simulink library "MK_SZ"  (R2026a)
settings: Solver=VariableStepAuto
settings Model: Creator=Szalay  LastModifiedBy=Szalay

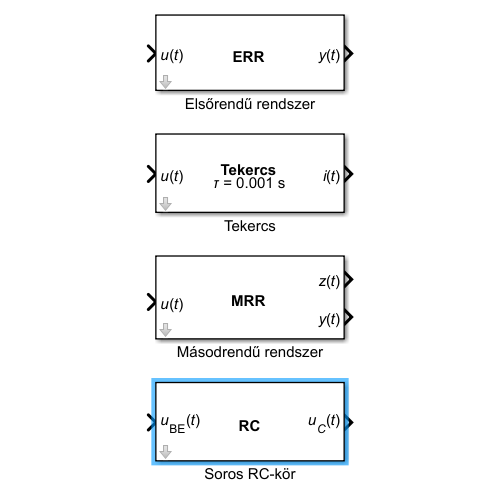
[thumbnail: Simulink's stored preview of the top-level diagram]
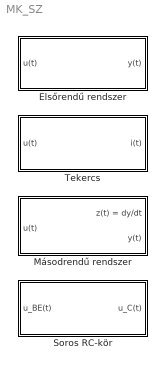
== system MK_SZ ==
  Elsőrendű rendszer : Subsystem  mask(Elsőrendű rendszer){K=1, tau=1, y_0=0}
      mask prompts: K "Állandósult állapoti erősítés"; tau "Időállandó (s)"; y_0 "A kimenet kezdeti értéke"
      mask help: A lineáris elsőrendű rendszer modellje.
      mask DialogControl ParameterGroupVar Prompt: Rendszerparaméterek
      mask DialogControl Container3 Prompt: Kezdeti érték
      mask Display:
      | % Csatlakozók
      | port_label('input', 1, '{\itu}({\itt})', 'texmode', 'on');
      | port_label('output', 1, '{\ity}({\itt})', 'texmode', 'on');
      | 
      | % Felirat
      | text(0.5, 0.5, '{\bfERR}', ...
      |     'HorizontalAlignment', 'center', ...
      |     'Interpreter', 'tex' ...
      |     );
  Másodrendű rendszer : Subsystem  mask(Másodrendű rendszer){K=1, tau=1, xi=1, y_0=0, z_0=0}
      mask prompts: K "Állandósult állapoti erősítés"; tau "Időállandó (s)"; xi "Csillapítási tényező"; y_0 "Kezdeti y"; z_0 "Kezdeti z"
      mask help: A közönséges lineáris másodfokú differenciálegyenlet megoldása.
      mask DialogControl ParameterGroupVar Prompt: Rendszerparaméterek
      mask DialogControl Container3 Prompt: Kezdeti értékek
      mask Display:
      | % Csatlakozók
      | port_label('input', 1, '{\itu}({\itt})', 'texmode', 'on');
      | port_label('output', 1, '{\itz}({\itt})', 'texmode', 'on');
      | port_label('output', 2, '{\ity}({\itt})', 'texmode', 'on');
      | 
      | % Felirat
      | text(0.5, 0.5, '{\bfMRR}', ...
      |     'HorizontalAlignment', 'center', ...
      |     'Interpreter', 'tex' ...
      |     );
  Soros RC-kör : Subsystem  mask(RC-kör){R=1, C=1e-6, u_C0=0}
      mask prompts: R "Ellenállás"; C "Kapacitás"; u_C0 "A kapacitás kezdeti feszültsége"
      mask help: A soros RC-kör modellje.
      mask DialogControl ParameterGroupVar Prompt: Modellparaméterek
      mask DialogControl Container3 Prompt: Kezdeti érték
      mask Display:
      | % Csatlakozók
      | port_label('input', 1, '{\itu}_{BE}({\itt})', 'texmode', 'on');
      | port_label('output', 1, '{\itu}_{\itC}({\itt})', 'texmode', 'on');
      | 
      | % Felirat
      | text(0.5, 0.5, '{\bfRC}', ...
      |     'HorizontalAlignment', 'center', ...
      |     'Interpreter', 'tex' ...
      |     );
  Tekercs : Subsystem  mask(Tekercs){R=1, L=1e-3, i_0=0}
      mask prompts: R "Ellenállás"; L "Öninduktivitás"; i_0 "Kezdeti áramerősség"
      mask help: Lineáris mágnesezésű tekercsmodell.
      mask DialogControl ParameterGroupVar Prompt: Modellparaméterek
      mask DialogControl Container3 Prompt: Kezdeti érték
      mask Display:
      | % Csatlakozók
      | port_label('input', 1, '{\itu}({\itt})', 'texmode', 'on');
      | port_label('output', 1, '{\iti}({\itt})', 'texmode', 'on');
      | 
      | R = str2double(get_param(gcb, 'R'));
      | L = str2double(get_param(gcb, 'L'));
      | 
      | tau = L/R;
      | 
      | % Felirat
      | text(0.5, 0.5, [ ...
      |     '{\bfTekercs}', newline, '{\it\tau} = ', sprintf('%g', tau), ' s' ...
      |     ], ...
      |     'HorizontalAlignment', 'center', ...
      |     'Interpreter', 'tex' ...
      |     );

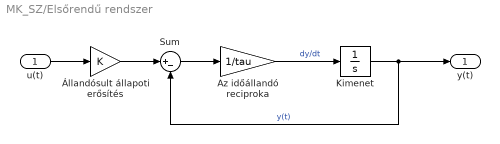
== system MK_SZ/Elsőrendű rendszer ==
  u(t) : Inport
  Az időállandó reciproka : Gain  Gain=1/tau
  Kimenet : Integrator  InitialCondition=y_0
  Sum : Sum  Inputs=|+-
  Állandósult állapoti erősítés : Gain  Gain=K
  y(t) : Outport
  wires:
  Kimenet/1 -> y(t)/1, Sum/2  "y(t)"
  Az időállandó reciproka/1 -> Kimenet/1  "dy/dt"
  Állandósult állapoti erősítés/1 -> Sum/1
  Sum/1 -> Az időállandó reciproka/1
  u(t)/1 -> Állandósult állapoti erősítés/1

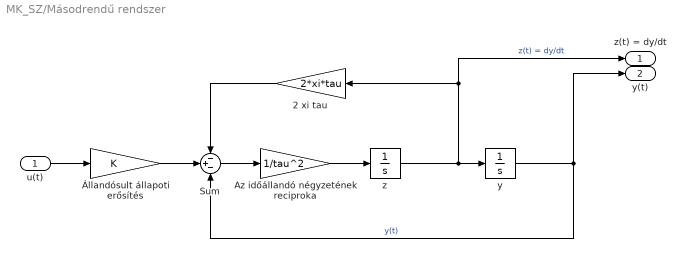
== system MK_SZ/Másodrendű rendszer ==
  u(t) : Inport
  2 xi tau : Gain  Gain=2*xi*tau
  Az időállandó négyzetének reciproka : Gain  Gain=1/tau^2
  Sum : Sum  Inputs=-+-
  y : Integrator  InitialCondition=y_0
  z : Integrator  InitialCondition=z_0
  Állandósult állapoti erősítés : Gain  Gain=K
  z(t) = dy/dt : Outport
  y(t) : Outport  Port=2
  wires:
  2 xi tau/1 -> Sum/1
  y/1 -> Sum/3, y(t)/1  "y(t)"
  Sum/1 -> Az időállandó négyzetének reciproka/1
  Az időállandó négyzetének reciproka/1 -> z/1
  z/1 -> y/1, 2 xi tau/1, z(t) = dy/dt/1  "z(t) = dy/dt"
  Állandósult állapoti erősítés/1 -> Sum/2
  u(t)/1 -> Állandósult állapoti erősítés/1

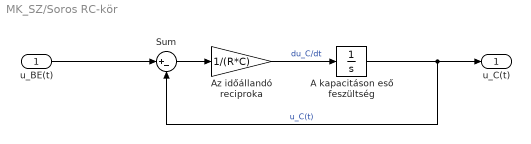
== system MK_SZ/Soros RC-kör ==
  u_BE(t) : Inport
  A kapacitáson eső feszültség : Integrator  InitialCondition=u_C0
  Az időállandó reciproka : Gain  Gain=1/(R*C)
  Sum : Sum  Inputs=|+-
  u_C(t) : Outport
  wires:
  Sum/1 -> Az időállandó reciproka/1
  A kapacitáson eső feszültség/1 -> Sum/2, u_C(t)/1  "u_C(t)"
  Az időállandó reciproka/1 -> A kapacitáson eső feszültség/1  "du_C/dt"
  u_BE(t)/1 -> Sum/1

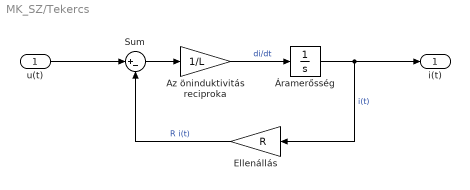
== system MK_SZ/Tekercs ==
  u(t) : Inport
  Az öninduktivitás reciproka : Gain  Gain=1/L
  Ellenállás : Gain  Gain=R
  Sum : Sum  Inputs=|+-
  Áramerősség : Integrator  InitialCondition=i_0
  i(t) : Outport
  wires:
  Az öninduktivitás reciproka/1 -> Áramerősség/1  "di/dt"
  Ellenállás/1 -> Sum/2  "R i(t)"
  Áramerősség/1 -> Ellenállás/1, i(t)/1  "i(t)"
  u(t)/1 -> Sum/1
  Sum/1 -> Az öninduktivitás reciproka/1
